simulink model "exo_df"  (R2018a)
settings: Solver=FixedStepDiscrete  StartTime=0.0  StopTime=inf  FixedStep=0.001  RelTol=1e-3  EnableMultiTasking=on
InitFcn:
  | init
values from neighbouring files (symbols this model uses):
  motor_saturation_torque = [10.0, 10.0]    [init.m]
  n = 2    [init.m]
  treadmillSpeed = 1.1    [init.m]
undefined symbols (not defined in the file or in its folder): DiscIntNeverNeededParam, Q8, USB
libraries: hdlsllib x50, quarc_library x16, dspsigops x2
(part 1 of 2)
settings Model: SimulationMode=external  ExtModeTrigDuration=2000000  Creator=mdmancho  LastModifiedBy=mdmancho
settings SolverCC: PositivePriorityOrder=on
settings RTWCC: SystemTargetFile=quarc_win64.tlc  TemplateMakefile=quarc_default_tmf  Description=QUARC Win64 Target
settings STFCustomTargetCC: TargetPreCompLibLocation=C:\PROGRA~3\QUARC\lib\2018a\win64\release  TargetLangStandard=C99 (ISO)  ConcurrentExecutionCompliant=on  SystemTargetFile=quarc_win64.tlc
settings GRTTargetCC: TargetPreCompLibLocation=C:\PROGRA~3\QUARC\lib\2018a\win64\release  ParMdlRefBuildCompliant=off  CompOptLevelCompliant=off  CombineOutputUpdateFcns=off  MatFileLogging=off  CPPClassGenCompliant=off  GRTInterface=on  UseToolchainInfoCompliant=off  ExtMode=on  ExtModeMexFile=quarc_comm

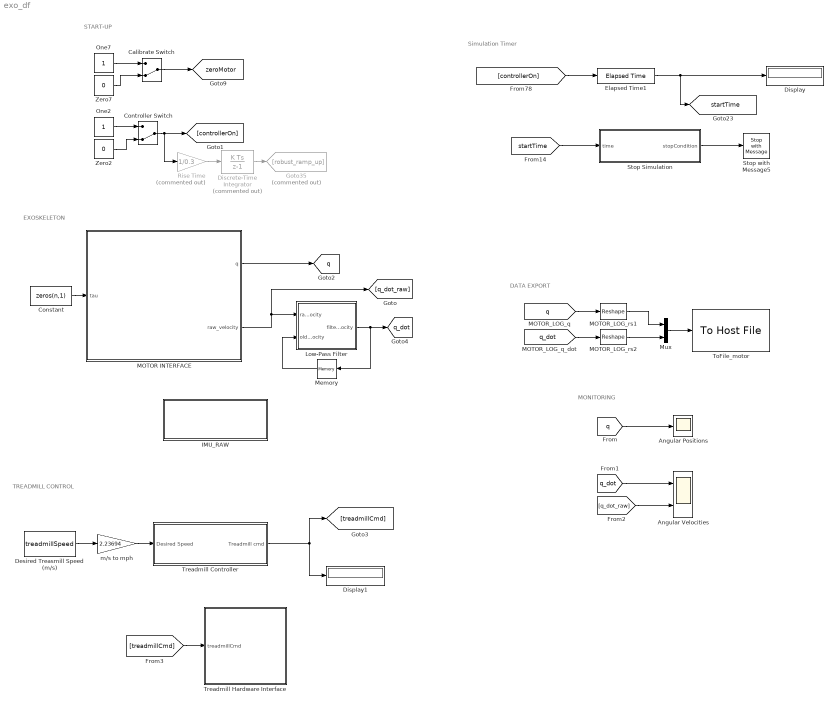
== system exo_df ==
  note: DATA EXPORT
  note: MONITORING
  note: START-UP
  note: EXOSKELETON
  note: Simulation Timer
  note: TREADMILL CONTROL
  Angular Positions : Scope
  Angular Velocities : Scope  NumInputPorts=2
  Calibrate Switch : ManualSwitch  CurrentSetting=0
  Constant : Constant  Value=zeros(n,1)
  Controller Switch : ManualSwitch  CurrentSetting=0
  Desired Treasmill Speed (m/s) : Constant  Value=treadmillSpeed
  Discrete-Time Integrator : DiscreteIntegrator  Commented=on  SampleTime=-1  LimitOutput=on  UpperSaturationLimit=1  LowerSaturationLimit=0  ICPrevOutput=DiscIntNeverNeededParam  ICPrevScaledInput=DiscIntNeverNeededParam
  Display : Display
  Display1 : Display
  Elapsed Time1 : quarc_library/Advanced/Timing/Elapsed Time  start_src=on
      settings: SourceProductName=QUARC Targets
  Goto35 : Goto  Commented=on  GotoTag=robust_ramp_up
  IMU_RAW : Subsystem  Description=Shoe VN-100 raw acquisition for OFFLINE validation only. No outports: nothing in the controller or the phase estimator may read it. See README.md.
  Low-Pass Filter : MATLAB Function  TreatAsAtomicUnit=on
  MOTOR INTERFACE : Subsystem
  MOTOR_LOG_rs1 : Reshape
  MOTOR_LOG_rs2 : Reshape
  Memory : quarc_library/Discrete/Memory  initial_condition=zeros(2,1)  sample_time=-1
      settings: SourceProductName=QUARC Targets
  Mux : Mux  Inputs=2
  One2 : Constant
  One7 : Constant
  Rise Time : Gain  Commented=on  Gain=1/0.3
  Stop Simulation : MATLAB Function  TreatAsAtomicUnit=on
  Stop with Message5 : quarc_library/Sinks/Error Handling/Stop with Message  message_type=Fixed error message  message_icon=Error  message=Simulation has ended
  ToFile_motor : quarc_library/Sinks/To Host/To Host File  file_name=C:\exo_logs\%{vn_log_run}_motor.mat  variable_name=motor  decimation=1  sample_time=-1  file_format=MAT-file v.5  options=No header or footer  append=off  final_file_name=C:\exo_logs\S02_T02_motor.mat  bitrate=2000000
  Treadmill Controller : Subsystem
  Treadmill Hardware Interface : Subsystem
  Zero2 : Constant  Value=0
  Zero7 : Constant  Value=0
  m/s to mph : Gain  Gain=2.23694
  tag scope: q=global, q_dot=global, startTime=global, zeroMotor=global
  wires:
  Memory/1 -> Low-Pass Filter/2(old_filtered_velocity)
  Low-Pass Filter/1(filtered_velocity) -> [q_dot], Memory/1
  MOTOR INTERFACE/2(raw_velocity) -> [q_dot_raw], Low-Pass Filter/1(raw_velocity)
  MOTOR INTERFACE/1(q) -> [q]
  [controllerOn] -> Elapsed Time1/1
  Elapsed Time1/1 -> Display/1, [startTime]
  Rise Time/1 -> Discrete-Time Integrator/1
  Discrete-Time Integrator/1 -> Goto35/1
  Calibrate Switch/1 -> [zeroMotor]
  Controller Switch/1 -> Rise Time/1, [controllerOn]
  One7/1 -> Calibrate Switch/1
  Zero2/1 -> Controller Switch/2
  Zero7/1 -> Calibrate Switch/2
  One2/1 -> Controller Switch/1
  Constant/1 -> MOTOR INTERFACE/1("tau ")
  [q] -> Angular Positions/1
  [q_dot] -> Angular Velocities/1
  [q_dot_raw] -> Angular Velocities/2
  [q] -> MOTOR_LOG_rs1/1
  [q_dot] -> MOTOR_LOG_rs2/1
  MOTOR_LOG_rs1/1 -> Mux/1
  MOTOR_LOG_rs2/1 -> Mux/2
  Mux/1 -> ToFile_motor/1
  [startTime] -> Stop Simulation/1(time)
  Stop Simulation/1(stopCondition) -> Stop with Message5/1
  [treadmillCmd] -> Treadmill Hardware Interface/1(treadmillCmd)
  Desired Treasmill Speed (m/s)/1 -> m/s to mph/1
  Treadmill Controller/1(Treadmill cmd) -> [treadmillCmd], Display1/1
  m/s to mph/1 -> Treadmill Controller/1(Desired Speed)

== system exo_df/IMU_RAW ==
  CLK : Subsystem
  RX : Subsystem

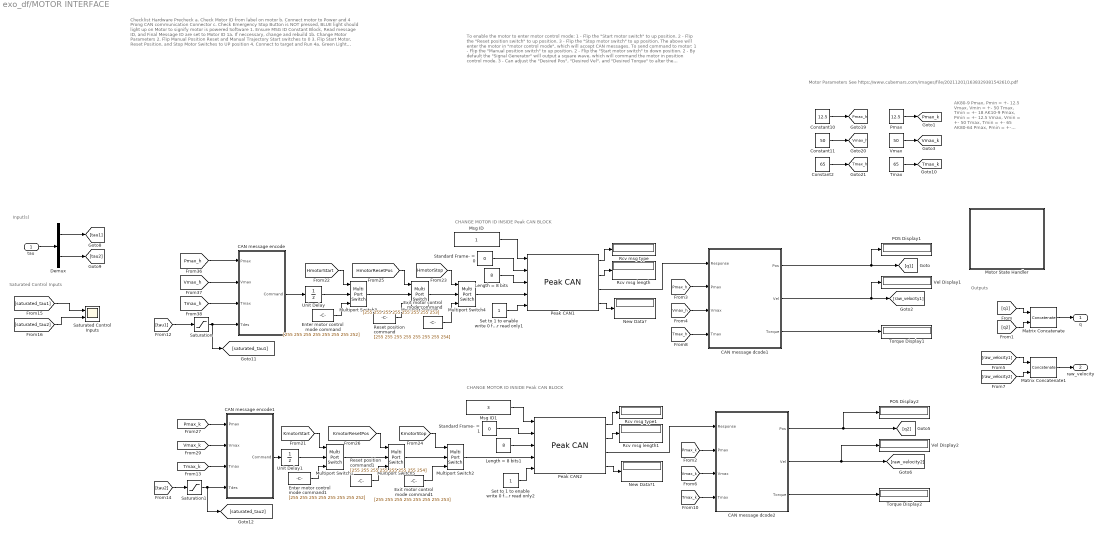
== system exo_df/MOTOR INTERFACE ==
  note: Saturated Control Inputs
  note: Input(s)
  note: Outputs
  note: CHANGE MOTOR ID INSIDE Peak CAN BLOCK
  note: Motor Parameters
      | See https://www.cubemars.com/images/file/20211201/1638329381542610.pdf
  note: To enable the motor to enter motor control mode:
      | 1 - Flip the "Start motor switch" to up position.
      | 2 - Flip the "Reset position switch" to up position.
      | 3 - Flip the "Stop motor switch" to up position.
      | The above will enter the motor in "motor control mode", which will accept CAN messages.
      |
      | To send command to motor:
      | 1 - Flip the "Manual position switch" to up position.
      | 2 - Flip the "Start motor switch" to down position.
      | 2 - By default the "Signal Generator" will output a square wave, which will command the motor in position control mode.
      | 3 - Can adjust the "Desired Pos", "Desired Vel", and "Desired Torque" to alter the command.
      | 4 - Can adjust the "Kp" and "Kd" to alter the P and D gain of the motor's internal controller.
      | 5 - If want to reset the motor position to 0, flip the "Reset position switch" to down position.
      |
      | To stop the motor and disable motor control mode:
      | 1 - Set the "Desired Pos", "Desired Vel", and "Desired Torque" to 0.
      | 2 - Flip the "Start motor switch" to up position.
      | 3 - Flip the "Stop motor switch" to down position.
  note: AK80-9
      | Pmax, Pmin = +- 12.5
      | Vmax, Vmin = +- 50
      | Tmax, Tmin = +- 18
      |
      | AK10-9
      | Pmax, Pmin = +- 12.5
      | Vmax, Vmin = +- 50
      | Tmax, Tmin = +- 65
      |
      | AK80-64
      | Pmax, Pmin = +- 12.5
      | Vmax, Vmin = +- 8
      | Tmax, Tmin = +- 144
  note: Checklist
      | Hardware Precheck
      | 	a. Check Motor ID from label on motor
      | 	b. Connect motor to Power and 4 Prong CAN communication Connector
      | 	c. Check Emergency Stop Button is NOT pressed, BLUE light should light up on Motor to 						signify motor is powered
      | Software
      | 1. Ensure MSG ID Constant Block, Read message ID, and Final Message ID are set to Motor ID
      | 	1a. If neccessary, change and rebuild
      | 	1b. Change Motor Parameters
      | 2. Flip Manual Position Reset and Manual Trajectory Start switches to 0
      | 3. Flip Start Motor, Reset Position, and Stop Motor Switches to UP position
      | 4. Connect to target and Run
      | 	4a. Green Light should light up on motor
      | 5. Flip Reset Position Switch to DOWN position, POS Display should now show a number (likely ~0 or ~-25)
      | 	5a. Flip Manual Position Offset switch, POS Display should now be 0
      | 	5b. Flip Reset Position Switch to UP position
      | 6. Flip Start Motor Switch to DOWN position
      | 7. Flip Manual Traj Start switch to 1
  note: CHANGE MOTOR ID INSIDE Peak CAN BLOCK
  "tau " : Inport
  CAN message dcode1 : Subsystem
  CAN message dcode2 : Subsystem
  CAN message encode : Subsystem
  CAN message encode1 : Subsystem
  Constant10 : Constant  Value=12.5
  Constant11 : Constant  Value=50
  Constant2 : Constant  Value=65
  Demux : Demux  Outputs=2
  Enter motor control mode command : Constant  Value=[255 255 255 255 255 255 255 252]  OutDataTypeStr=uint8
  Enter motor control mode command1 : Constant  Value=[255 255 255 255 255 255 255 252]  OutDataTypeStr=uint8
  Exit motor control mode command : Constant  Value=[255 255 255 255 255 255 255 253]  OutDataTypeStr=uint8
  Exit motor control mode command1 : Constant  Value=[255 255 255 255 255 255 255 253]  OutDataTypeStr=uint8
  Length = 8 bits : Constant  Value=8  OutDataTypeStr=uint8
  Length = 8 bits1 : Constant  Value=8  OutDataTypeStr=uint8
  Matrix Concatenate : Concatenate  Mode=Multidimensional array
  Matrix Concatenate1 : Concatenate  Mode=Multidimensional array
  Motor State Handler : Subsystem
  Msg ID : Constant  OutDataTypeStr=uint32
  Msg ID1 : Constant  Value=3  OutDataTypeStr=uint32
  Multiport Switch{1..6} (6 alike) : MultiPortSwitch  Inputs=2
  New Data? : Display
  New Data?1 : Display
  POS Display1 : Display
      settings: Format=decimal (Stored Integer)
  POS Display2 : Display
      settings: Format=decimal (Stored Integer)
  Peak CAN1 : quarc_library/Devices/Third-Party/Peak System/CAN Interfaces/Peak CAN  channel=2  device_type=PCAN-USB and PCAN-USB Pro  baud=1 Mbit/s  msg_ids=1  rcv_thread=off  thread_priority=0  send_final_message=on  final_id=1  final_type=0  final_data=[255 255 255 255 255 255 255 253]  sample_time=qc_get_step_size
      settings: SourceProductName=QUARC Targets
  Peak CAN2 : quarc_library/Devices/Third-Party/Peak System/CAN Interfaces/Peak CAN  channel=1  device_type=PCAN-USB and PCAN-USB Pro  baud=1 Mbit/s  msg_ids=3  rcv_thread=off  thread_priority=0  send_final_message=on  final_id=3  final_type=0  final_data=[255 255 255 255 255 255 255 253]  sample_time=qc_get_step_size
      settings: SourceProductName=QUARC Targets
  Pmax : Constant  Value=12.5
  Rcv msg length : Display
  Rcv msg length1 : Display
  Rcv msg type : Display
  Rcv msg type1 : Display
  Reset position command : Constant  Value=[255 255 255 255 255 255 255 254]  OutDataTypeStr=uint8
  Reset position command1 : Constant  Value=[255 255 255 255 255 255 255 254]  OutDataTypeStr=uint8
  Saturated Control Inputs : Scope  NumInputPorts=2
  Saturation : Saturate  UpperLimit=motor_saturation_torque(1)  LowerLimit=-motor_saturation_torque(1)
  Saturation1 : Saturate  UpperLimit=motor_saturation_torque(2)  LowerLimit=-motor_saturation_torque(2)
  Set to 1 to enable write 0 for read only1 : Constant  OutDataTypeStr=boolean
  Set to 1 to enable write 0 for read only2 : Constant  OutDataTypeStr=boolean
  Standard Frame- = 0 : Constant  Value=0  OutDataTypeStr=uint8
  Standard Frame- = 1 : Constant  Value=0  OutDataTypeStr=uint8
  Tmax : Constant  Value=65
  Torque Display1 : Display
      settings: Format=decimal (Stored Integer)
  Torque Display2 : Display
      settings: Format=decimal (Stored Integer)
  Unit Delay : UnitDelay  SampleTime=-1
  Unit Delay1 : UnitDelay  SampleTime=-1
  Vel Display1 : Display
      settings: Format=decimal (Stored Integer)
  Vel Display2 : Display
      settings: Format=decimal (Stored Integer)
  Vmax : Constant  Value=50
  q : Outport
  raw_velocity : Outport  Port=2
  tag scope: Pmax_h=global, Pmax_k=global, Tmax_h=global, Tmax_k=global, Vmax_h=global, Vmax_k=global
  wires:
  [Vmax_h] -> CAN message dcode1/3(Vmax)
  Saturation/1 -> [saturated_tau1], CAN message encode/4(Tdes)
  Length = 8 bits1/1 -> Peak CAN2/3
  Enter motor control mode command/1 -> Multiport Switch3/3
  [KmotorStart] -> Multiport Switch1/1
  [Pmax_h] -> CAN message encode/1(Pmax)
  Multiport Switch6/1 -> Multiport Switch4/2
  Msg ID1/1 -> Peak CAN2/1
  Peak CAN2/1 -> Rcv msg type1/1
  Multiport Switch2/1 -> Peak CAN2/4
  CAN message encode1/1(Command) -> Unit Delay1/1
  [HmotorStop] -> Multiport Switch4/1
  Unit Delay1/1 -> Multiport Switch1/2
  [Tmax_k] -> CAN message encode1/3(Tmax)
  Peak CAN2/4 -> New Data?1/1
  Multiport Switch4/1 -> Peak CAN1/4
  [Vmax_k] -> CAN message encode1/2(Vmax)
  [HmotorResetPos] -> Multiport Switch6/1
  Standard Frame- = 1/1 -> Peak CAN2/2
  Exit motor control mode command/1 -> Multiport Switch4/3
  Saturation1/1 -> [saturated_tau2], CAN message encode1/4(Tdes)
  [Tmax_h] -> CAN message dcode1/4(Tmax)
  Msg ID/1 -> Peak CAN1/1
  Peak CAN1/2 -> Rcv msg length/1
  Peak CAN1/1 -> Rcv msg type/1
  Multiport Switch3/1 -> Multiport Switch6/2
  [HmotorStart] -> Multiport Switch3/1
  [Tmax_h] -> CAN message encode/3(Tmax)
  Reset position command/1 -> Multiport Switch6/3
  Length = 8 bits/1 -> Peak CAN1/3
  Reset position command1/1 -> Multiport Switch5/3
  Unit Delay/1 -> Multiport Switch3/2
  Multiport Switch5/1 -> Multiport Switch2/2
  Standard Frame- = 0/1 -> Peak CAN1/2
  Peak CAN1/4 -> New Data?/1
  Peak CAN2/2 -> Rcv msg length1/1
  [Vmax_k] -> CAN message dcode2/3(Vmax)
  Multiport Switch1/1 -> Multiport Switch5/2
  Peak CAN1/3 -> CAN message dcode1/1(Response)
  CAN message encode/1(Command) -> Unit Delay/1
  Exit motor control mode command1/1 -> Multiport Switch2/3
  [Pmax_h] -> CAN message dcode1/2(Pmax)
  [KmotorResetPos] -> Multiport Switch5/1
  Enter motor control mode command1/1 -> Multiport Switch1/3
  [Vmax_h] -> CAN message encode/2(Vmax)
  [KmotorStop] -> Multiport Switch2/1
  [Pmax_k] -> CAN message dcode2/2(Pmax)
  Peak CAN2/3 -> CAN message dcode2/1(Response)
  [Tmax_k] -> CAN message dcode2/4(Tmax)
  [Pmax_k] -> CAN message encode1/1(Pmax)
  Set to 1 to enable write 0 for read only2/1 -> Peak CAN2/5
  Set to 1 to enable write 0 for read only1/1 -> Peak CAN1/5
  CAN message dcode1/1(Pos) -> [q1], POS Display1/1
  CAN message dcode1/2(Vel) -> [raw_velocity1], Vel Display1/1
  CAN message dcode2/1(Pos) -> [q2], POS Display2/1
  CAN message dcode2/2(Vel) -> [raw_velocity2], Vel Display2/1
  Constant10/1 -> [Pmax_h]
  Constant2/1 -> [Tmax_h]
  Vmax/1 -> [Vmax_k]
  Pmax/1 -> [Pmax_k]
  Constant11/1 -> [Vmax_h]
  Tmax/1 -> [Tmax_k]
  CAN message dcode2/3(Torque) -> Torque Display2/1
  CAN message dcode1/3(Torque) -> Torque Display1/1
  Matrix Concatenate/1 -> q/1
  [tau1] -> Saturation/1
  [tau2] -> Saturation1/1
  "tau "/1 -> Demux/1
  Demux/1 -> [tau1]
  Demux/2 -> [tau2]
  [q1] -> Matrix Concatenate/1
  [q2] -> Matrix Concatenate/2
  [raw_velocity1] -> Matrix Concatenate1/1
  [raw_velocity2] -> Matrix Concatenate1/2
  Matrix Concatenate1/1 -> raw_velocity/1
  [saturated_tau1] -> Saturated Control Inputs/1
  [saturated_tau2] -> Saturated Control Inputs/2

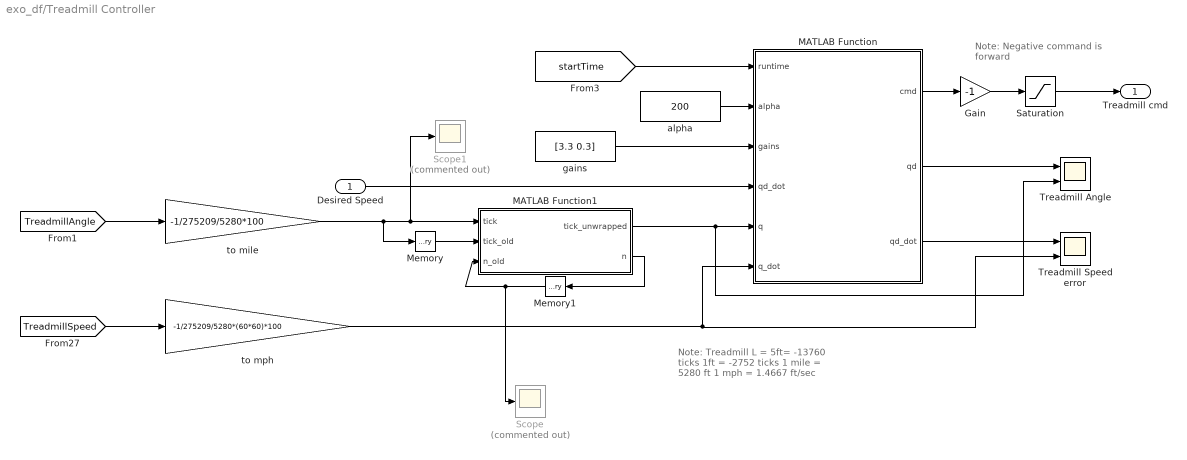
== system exo_df/Treadmill Controller ==
  note: Note:
      | Treadmill L = 5ft= -13760 ticks
      | 1ft = -2752 ticks
      | 1 mile = 5280 ft
      | 1 mph = 1.4667 ft/sec
  note: Note:
      | Negative command is forward
  Desired Speed : Inport
  Gain : Gain  Gain=-1
  MATLAB Function : MATLAB Function  TreatAsAtomicUnit=on
  MATLAB Function1 : MATLAB Function  TreatAsAtomicUnit=on
  Memory : Memory
  Memory1 : Memory
  Saturation : Saturate  UpperLimit=0  LowerLimit=-2
  Scope : Scope  Commented=on
  Scope1 : Scope  Commented=on
  Treadmill Angle : Scope  NumInputPorts=2
  Treadmill Speed error : Scope  NumInputPorts=2
  alpha : Constant  Value=200
  gains : Constant  Value=[3.3 0.3]
  to mile : Gain  Gain=-1/275209/5280*100
  to mph : Gain  Gain=-1/275209/5280*(60*60)*100
  Treadmill cmd : Outport
  wires:
  [TreadmillSpeed] -> to mph/1
  Saturation/1 -> Treadmill cmd/1
  to mph/1 -> Treadmill Speed error/2, MATLAB Function/6(q_dot)
  [startTime] -> MATLAB Function/1(runtime)
  gains/1 -> MATLAB Function/3(gains)
  MATLAB Function/1(cmd) -> Gain/1
  Desired Speed/1 -> MATLAB Function/4("qd_dot ")
  Gain/1 -> Saturation/1
  MATLAB Function/2(qd) -> Treadmill Angle/1
  MATLAB Function/3(qd_dot) -> Treadmill Speed error/1
  alpha/1 -> MATLAB Function/2(alpha)
  [TreadmillAngle] -> to mile/1
  Memory/1 -> MATLAB Function1/2(tick_old)
  MATLAB Function1/2(n) -> Memory1/1
  Memory1/1 -> Scope/1, MATLAB Function1/3(n_old)
  to mile/1 -> Memory/1, Scope1/1, MATLAB Function1/1(tick)
  MATLAB Function1/1(tick_unwrapped) -> Treadmill Angle/2, MATLAB Function/5(q)

== system exo_df/Treadmill Hardware Interface ==
  treadmillCmd : Inport
  Discrete Second-Order Low-Pass Filter2 : quarc_library/Discrete/Discrete Second-Order Low-Pass Filter  params_source=Internal (dialog parameters)  input_width=30  input_zeta=1  input_init=0  sample_time=sample_time
      settings: SourceProductName=QUARC Targets
  HIL Initialize : quarc_library/Data Acquisition/Generic/Configuration/HIL Initialize  Commented=on  object_name=QPID_e  board_type=qpid_e  board_number=0  board_options=enc0_dir=0;enc0_filter=1;enc0_a=1;enc0_b=1;enc0_z=0;enc0_reload=0;enc1_dir=0;enc1_filter=1;enc1_a=1;enc1_b=1;enc1_z=0;enc1_reload=0;enc2_dir=0;enc2_filter=1;enc2_a=1;enc2_b=1;enc2_z=0;enc2_reload=0;enc3_dir=0;enc3_filter=1;enc3_a=1;enc3_b=1;enc3_z=0;enc3_reload=0;enc4_dir=0;enc4_filter=1;enc4_a=1;enc4_b=1;enc4_z=0;enc4_reload=0;enc5_dir=0;enc5_filter=1;enc5_a=1;enc5_b=1;enc5_z=0;enc5_reload=0;enc6_dir=0;enc6_filter=1;enc6_a=1;enc6_b=1;enc6_z=0;enc6_reload=0;enc7_dir=0;enc7_filter=1;enc7_a=1;enc7_b=1;enc7_z=0;enc7_reload=0;ext_int_polarity=0;fuse_polarity=0;convert_polarity=0;watchdog_polarity=0;ext_int_watchdog=0;fuse_watchdog=0;trig1_watchdog=0;watchdog_to_trig1=0;watchdog_to_trig2=0;counter_to_trig0=0;trigger_adcs=0;latch_on_adc=0;pwm_immediate=0  exclusive=off  active=on  hardware_clocks=[0:16]  clock_modes=[]  initial_clock_frequencies=[]  set_clock_params_at_start=off  set_clock_params_at_switch_in=off  set_clock_frequencies_at_start=off  set_clock_frequencies_at_switch_in=off  analog_input_channels=[0:7]  analog_input_configurations=[]  analog_input_maximums=10  analog_input_minimums=-10  set_analog_input_params_at_start=off  set_analog_input_params_at_switch_in=off  analog_output_channels=[0:7]  analog_output_maximums=10  analog_output_minimums=-10  initial_analog_outputs=[0]  final_analog_outputs=[0]  watchdog_analog_outputs=0  set_analog_output_params_at_start=off  set_analog_output_params_at_switch_in=off  set_analog_outputs_at_start=on  set_analog_outputs_at_switch_in=off  set_analog_outputs_at_terminate=on  set_analog_outputs_at_switch_out=off  set_analog_outputs_on_watchdog=off  digital_input_channels=[]  digital_output_channels=[0:15]  digital_output_configuration=[]  initial_digital_outputs=[1]  final_digital_outputs=[1]  watchdog_digital_outputs=[2]  set_digital_output_params_at_start=off  set_digital_output_params_at_switch_in=off  set_digital_outputs_at_start=on  set_digital_outputs_at_switch_in=off  set_digital_outputs_at_terminate=on  set_digital_outputs_at_switch_out=off  set_digital_outputs_on_watchdog=off  encoder_channels=[0:7]  quadrature=[4]  encoder_filter_frequency=40e6/1  initial_encoder_counts=[0]  set_encoder_params_at_start=on  set_encoder_params_at_switch_in=off  set_encoder_counts_at_start=on  set_encoder_counts_at_switch_in=off  pwm_channels=[0:7]  pwm_modes=0  pwm_frequency=40e6/4096  pwm_configuration=[0]  pwm_alignment=[0]  pwm_polarity=[1]  pwm_leading_deadband=[0]  pwm_trailing_deadband=[0]  initial_pwm_outputs=[0]  final_pwm_outputs=[0]  watchdog_pwm_outputs=[0]  set_pwm_params_at_start=on  set_pwm_params_at_switch_in=off  set_pwm_outputs_at_start=on  set_pwm_outputs_at_switch_in=off  set_pwm_outputs_at_terminate=on  set_pwm_outputs_at_switch_out=off  set_pwm_outputs_on_watchdog=off  other_output_channels=[]  initial_other_outputs=[]  final_other_outputs=[]  watchdog_other_outputs=[]  set_other_outputs_at_start=off  set_other_outputs_at_switch_in=off  set_other_outputs_at_terminate=off  set_other_outputs_at_switch_out=off  set_other_outputs_on_watchdog=off
  HIL Initialize1 : quarc_library/Data Acquisition/Generic/Configuration/HIL Initialize  object_name=Q8-USB  board_type=q8_usb  board_number=0  board_options=update_rate=normal;decimation=1  exclusive=off  active=on  hardware_clocks=[0:2]  clock_modes=[]  initial_clock_frequencies=[]  set_clock_params_at_start=off  set_clock_params_at_switch_in=off  set_clock_frequencies_at_start=off  set_clock_frequencies_at_switch_in=off  analog_input_channels=[0:7]  analog_input_configurations=[]  analog_input_maximums=10  analog_input_minimums=-10  set_analog_input_params_at_start=on  set_analog_input_params_at_switch_in=off  analog_output_channels=[0:7]  analog_output_maximums=10  analog_output_minimums=-10  initial_analog_outputs=[0]  final_analog_outputs=[0]  watchdog_analog_outputs=0  set_analog_output_params_at_start=on  set_analog_output_params_at_switch_in=off  set_analog_outputs_at_start=on  set_analog_outputs_at_switch_in=off  set_analog_outputs_at_terminate=on  set_analog_outputs_at_switch_out=off  set_analog_outputs_on_watchdog=off  digital_input_channels=[]  digital_output_channels=[0]  digital_output_configuration=[]  initial_digital_outputs=[1]  final_digital_outputs=[1]  watchdog_digital_outputs=[0]  set_digital_output_params_at_start=off  set_digital_output_params_at_switch_in=off  set_digital_outputs_at_start=on  set_digital_outputs_at_switch_in=off  set_digital_outputs_at_terminate=on  set_digital_outputs_at_switch_out=off  set_digital_outputs_on_watchdog=off  encoder_channels=[0:7]  quadrature=[4]  encoder_filter_frequency=[]  initial_encoder_counts=[0]  set_encoder_params_at_start=on  set_encoder_params_at_switch_in=off  set_encoder_counts_at_start=on  set_encoder_counts_at_switch_in=off  pwm_channels=[0:7]  pwm_modes=0  pwm_frequency=99.532799999999995e6/4095  pwm_configuration=[0]  pwm_alignment=[0]  pwm_polarity=[1]  pwm_leading_deadband=[0]  pwm_trailing_deadband=[0]  initial_pwm_outputs=[0]  final_pwm_outputs=[0]  watchdog_pwm_outputs=[0]  set_pwm_params_at_start=on  set_pwm_params_at_switch_in=off  set_pwm_outputs_at_start=on  set_pwm_outputs_at_switch_in=off  set_pwm_outputs_at_terminate=on  set_pwm_outputs_at_switch_out=off  set_pwm_outputs_on_watchdog=off  other_output_channels=[]  initial_other_outputs=[]  final_other_outputs=[]  watchdog_other_outputs=[]  set_other_outputs_at_start=off  set_other_outputs_at_switch_in=off  set_other_outputs_at_terminate=off  set_other_outputs_at_switch_out=off  set_other_outputs_on_watchdog=off
  HIL Read2 : quarc_library/Data Acquisition/Generic/Immediate I//O/HIL Read  object_name=Q8-USB  analog_channels=[]  encoder_channels=[0]  digital_channels=[]  other_channels=[14000]  sample_time=sample_time  active=on  vector_output=off  data_type_mode=Inherit via back propagation  encoder_data_type=double  digital_data_type=boolean
  HIL Write : quarc_library/Data Acquisition/Generic/Immediate I//O/HIL Write  object_name=Q8-USB  analog_channels=0  pwm_channels=[]  digital_channels=[]  other_channels=[]  sample_time=sample_time  active=off  vector_input=off
  Motor Cmd to Quanser : Scope  NumInputPorts=2
  Scope : Scope
  tag scope: TreadmillAngle=global, TreadmillSpeed=global
  wires:
  Discrete Second-Order Low-Pass Filter2/1 -> [TreadmillSpeed]
  HIL Read2/2 -> Discrete Second-Order Low-Pass Filter2/1
  HIL Read2/1 -> [TreadmillAngle]
  [TreadmillAngle] -> Motor Cmd to Quanser/1
  [TreadmillSpeed] -> Motor Cmd to Quanser/2
  treadmillCmd/1 -> Scope/1, HIL Write/1

== system exo_df/IMU_RAW/CLK ==
  ToFile_clk : quarc_library/Sinks/To Host/To Host File  file_name=C:\exo_logs\%{vn_log_run}_clk.mat  variable_name=clk  decimation=1  sample_time=-1  file_format=MAT-file v.5  options=No header or footer  append=off  final_file_name=C:\exo_logs\S02_T02_clk.mat  bitrate=2000000
  qpc_clock : S-Function  FunctionName=qpc_clock  Parameters=0.001  SFunctionDeploymentMode=off  EnableBusSupport=off
  wires:
  qpc_clock/1 -> ToFile_clk/1  "qpc_s"

== system exo_df/IMU_RAW/RX ==
  DTC{2..8} (7 alike) : DataTypeConversion  OutDataTypeStr=double
  Mux : Mux  Inputs=7
  Term_bytes : Terminator
  ToFile_bytes : quarc_library/Sinks/To Host/To Host File  file_name=C:\exo_logs\%{vn_log_run}_imu_bytes.mat  variable_name=imu_bytes_p4  decimation=1  sample_time=-1  file_format=MAT-file v.5  options=No header or footer  append=off  final_file_name=C:\exo_logs\S02_T02_imu_bytes.mat  bitrate=2000000
  ToFile_diag : quarc_library/Sinks/To Host/To Host File  file_name=C:\exo_logs\%{vn_log_run}_imu_diag.mat  variable_name=imu_diag  decimation=1  sample_time=-1  file_format=MAT-file v.5  options=No header or footer  append=off  final_file_name=C:\exo_logs\S02_T02_imu_diag.mat  bitrate=2000000
  vn_raw_rx : S-Function  FunctionName=vn_raw_rx  Parameters=9, 921600, 0.002, 128  SFunctionDeploymentMode=off  EnableBusSupport=off
  wires:
  vn_raw_rx/1 -> Term_bytes/1  "imu_bytes"
  vn_raw_rx/9 -> ToFile_bytes/1  "imu_bytes_p4"
  vn_raw_rx/2 -> DTC2/1  "n_read"
  DTC2/1 -> Mux/1
  vn_raw_rx/3 -> DTC3/1  "t_rx_qpc"
  DTC3/1 -> Mux/2
  vn_raw_rx/4 -> DTC4/1  "queued"
  DTC4/1 -> Mux/3
  vn_raw_rx/5 -> DTC5/1  "cum_bytes"
  DTC5/1 -> Mux/4
  vn_raw_rx/6 -> DTC6/1  "err_calls"
  DTC6/1 -> Mux/5
  vn_raw_rx/7 -> DTC7/1  "err_mask"
  DTC7/1 -> Mux/6
  vn_raw_rx/8 -> DTC8/1  "dur_us"
  DTC8/1 -> Mux/7
  Mux/1 -> ToFile_diag/1

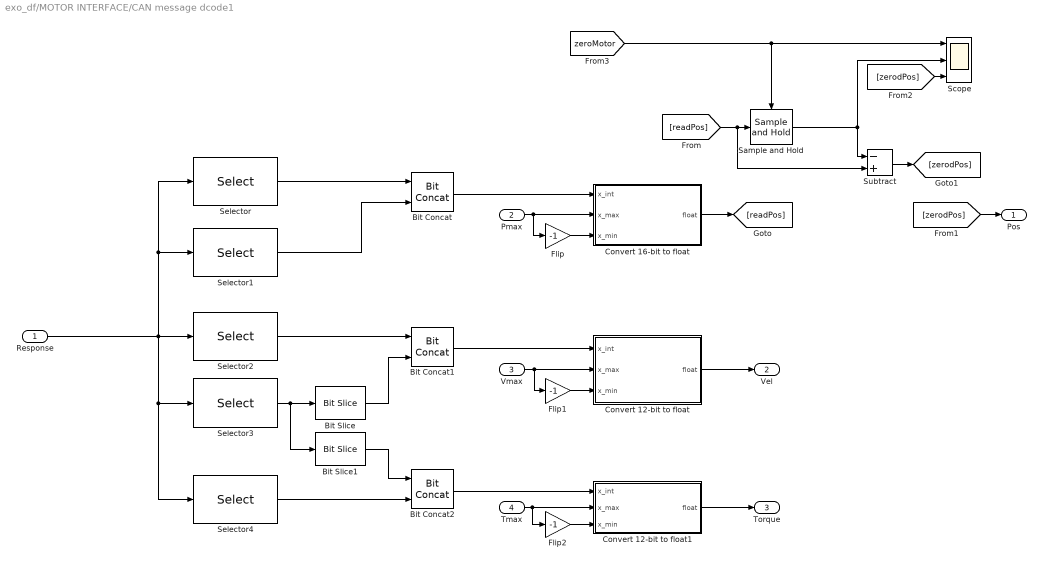
== system exo_df/MOTOR INTERFACE/CAN message dcode1 ==
  Response : Inport
  Pmax : Inport  Port=2
  Vmax : Inport  Port=3
  Tmax : Inport  Port=4
  Bit Concat : hdlsllib/Logic and Bit Operations/Bit Concat  numInputs=2
      settings: SourceProductName=HDL Coder  SourceProductBaseCode=HD
  Bit Concat1 : hdlsllib/Logic and Bit Operations/Bit Concat  numInputs=2
      settings: SourceProductName=HDL Coder  SourceProductBaseCode=HD
  Bit Concat2 : hdlsllib/Logic and Bit Operations/Bit Concat  numInputs=2
      settings: SourceProductName=HDL Coder  SourceProductBaseCode=HD
  Bit Slice : hdlsllib/Logic and Bit Operations/Bit Slice  lidx=7  ridx=4
  Bit Slice1 : hdlsllib/Logic and Bit Operations/Bit Slice  lidx=3  ridx=0
  Convert 12-bit to float : Subsystem
  Convert 12-bit to float1 : Subsystem
  Convert 16-bit to float : Subsystem
  Flip : Gain  Gain=-1
  Flip1 : Gain  Gain=-1
  Flip2 : Gain  Gain=-1
  Sample and Hold : dspsigops/Sample and Hold  trig=Rising edge  initCond=0  latchinput=off
  Scope : Scope  NumInputPorts=3
  Selector : Selector  IndexMode=Zero-based  InputPortWidth=8  IndexOptions=Index vector (dialog)  Indices=[1]  OutputSizes=1
  Selector1 : Selector  IndexMode=Zero-based  InputPortWidth=8  IndexOptions=Index vector (dialog)  Indices=[2]  OutputSizes=1
  Selector2 : Selector  IndexMode=Zero-based  InputPortWidth=8  IndexOptions=Index vector (dialog)  Indices=[3]  OutputSizes=1
  Selector3 : Selector  IndexMode=Zero-based  InputPortWidth=8  IndexOptions=Index vector (dialog)  Indices=[4]  OutputSizes=1
  Selector4 : Selector  IndexMode=Zero-based  InputPortWidth=8  IndexOptions=Index vector (dialog)  Indices=[5]  OutputSizes=1
  Subtract : Sum  Inputs=-+
  Pos : Outport  VectorParamsAs1DForOutWhenUnconnected=on
  Vel : Outport  Port=2  VectorParamsAs1DForOutWhenUnconnected=on
  Torque : Outport  Port=3  VectorParamsAs1DForOutWhenUnconnected=on
  wires:
  Vmax/1 -> Flip1/1, Convert 12-bit to float/2(x_max)
  Selector3/1 -> Bit Slice1/1, Bit Slice/1
  Bit Slice1/1 -> Bit Concat2/1
  Response/1 -> Selector4/1, Selector3/1, Selector/1, Selector1/1, Selector2/1
  Selector/1 -> Bit Concat/1
  Bit Concat2/1 -> Convert 12-bit to float1/1(x_int)
  Selector1/1 -> Bit Concat/2
  Pmax/1 -> Flip/1, Convert 16-bit to float/2(x_max)
  Bit Concat/1 -> Convert 16-bit to float/1(x_int)
  Selector2/1 -> Bit Concat1/1
  Selector4/1 -> Bit Concat2/2
  Flip1/1 -> Convert 12-bit to float/3(x_min)
  Tmax/1 -> Flip2/1, Convert 12-bit to float1/2(x_max)
  Bit Concat1/1 -> Convert 12-bit to float/1(x_int)
  Flip/1 -> Convert 16-bit to float/3(x_min)
  Bit Slice/1 -> Bit Concat1/2
  Convert 12-bit to float1/1(float) -> Torque/1
  Flip2/1 -> Convert 12-bit to float1/3(x_min)
  Convert 16-bit to float/1(float) -> [readPos]
  [readPos] -> Subtract/2, Sample and Hold/1
  Sample and Hold/1 -> Subtract/1, Scope/2
  Subtract/1 -> [zerodPos]
  [zerodPos] -> Pos/1
  [zerodPos] -> Scope/3
  [zeroMotor] -> Sample and Hold/Trigger, Scope/1
  Convert 12-bit to float/1(float) -> Vel/1

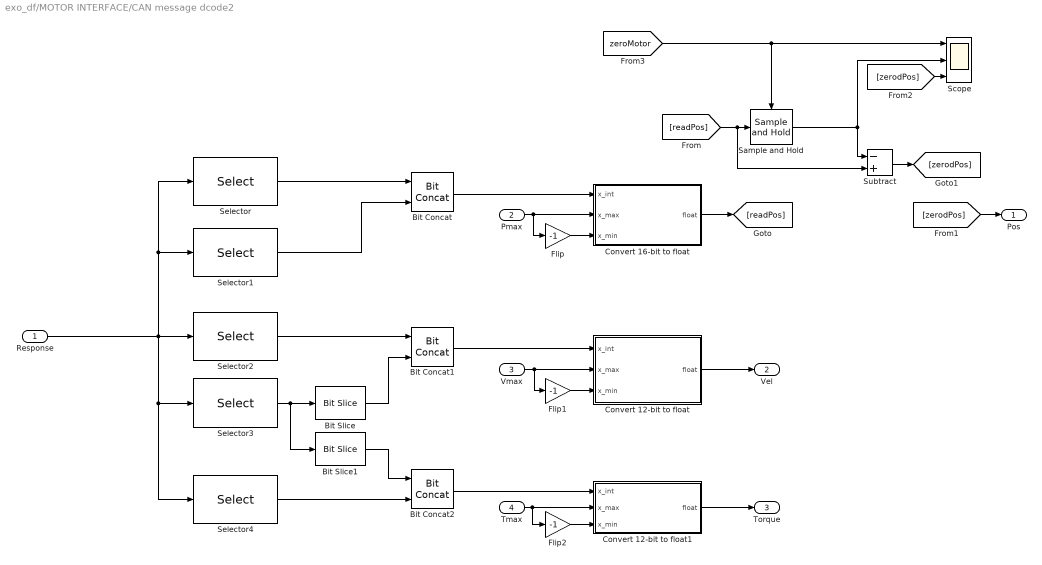
== system exo_df/MOTOR INTERFACE/CAN message dcode2 ==
  Response : Inport
  Pmax : Inport  Port=2
  Vmax : Inport  Port=3
  Tmax : Inport  Port=4
  Bit Concat : hdlsllib/Logic and Bit Operations/Bit Concat  numInputs=2
      settings: SourceProductName=HDL Coder  SourceProductBaseCode=HD
  Bit Concat1 : hdlsllib/Logic and Bit Operations/Bit Concat  numInputs=2
      settings: SourceProductName=HDL Coder  SourceProductBaseCode=HD
  Bit Concat2 : hdlsllib/Logic and Bit Operations/Bit Concat  numInputs=2
      settings: SourceProductName=HDL Coder  SourceProductBaseCode=HD
  Bit Slice : hdlsllib/Logic and Bit Operations/Bit Slice  lidx=7  ridx=4
  Bit Slice1 : hdlsllib/Logic and Bit Operations/Bit Slice  lidx=3  ridx=0
  Convert 12-bit to float : Subsystem
  Convert 12-bit to float1 : Subsystem
  Convert 16-bit to float : Subsystem
  Flip : Gain  Gain=-1
  Flip1 : Gain  Gain=-1
  Flip2 : Gain  Gain=-1
  Sample and Hold : dspsigops/Sample and Hold  trig=Rising edge  initCond=0  latchinput=off
  Scope : Scope  NumInputPorts=3
  Selector : Selector  IndexMode=Zero-based  InputPortWidth=8  IndexOptions=Index vector (dialog)  Indices=[1]  OutputSizes=1
  Selector1 : Selector  IndexMode=Zero-based  InputPortWidth=8  IndexOptions=Index vector (dialog)  Indices=[2]  OutputSizes=1
  Selector2 : Selector  IndexMode=Zero-based  InputPortWidth=8  IndexOptions=Index vector (dialog)  Indices=[3]  OutputSizes=1
  Selector3 : Selector  IndexMode=Zero-based  InputPortWidth=8  IndexOptions=Index vector (dialog)  Indices=[4]  OutputSizes=1
  Selector4 : Selector  IndexMode=Zero-based  InputPortWidth=8  IndexOptions=Index vector (dialog)  Indices=[5]  OutputSizes=1
  Subtract : Sum  Inputs=-+
  Pos : Outport  VectorParamsAs1DForOutWhenUnconnected=on
  Vel : Outport  Port=2  VectorParamsAs1DForOutWhenUnconnected=on
  Torque : Outport  Port=3  VectorParamsAs1DForOutWhenUnconnected=on
  wires:
  [zerodPos] -> Scope/3
  [zerodPos] -> Pos/1
  Subtract/1 -> [zerodPos]
  Sample and Hold/1 -> Scope/2, Subtract/1
  [readPos] -> Sample and Hold/1, Subtract/2
  Convert 16-bit to float/1(float) -> [readPos]
  Flip2/1 -> Convert 12-bit to float1/3(x_min)
  Convert 12-bit to float1/1(float) -> Torque/1
  Bit Slice/1 -> Bit Concat1/2
  Flip/1 -> Convert 16-bit to float/3(x_min)
  Bit Concat1/1 -> Convert 12-bit to float/1(x_int)
  Tmax/1 -> Convert 12-bit to float1/2(x_max), Flip2/1
  Flip1/1 -> Convert 12-bit to float/3(x_min)
  Selector4/1 -> Bit Concat2/2
  Selector2/1 -> Bit Concat1/1
  Bit Concat/1 -> Convert 16-bit to float/1(x_int)
  Pmax/1 -> Convert 16-bit to float/2(x_max), Flip/1
  Selector1/1 -> Bit Concat/2
  Bit Concat2/1 -> Convert 12-bit to float1/1(x_int)
  Selector/1 -> Bit Concat/1
  Response/1 -> Selector2/1, Selector1/1, Selector/1, Selector3/1, Selector4/1
  Bit Slice1/1 -> Bit Concat2/1
  Selector3/1 -> Bit Slice/1, Bit Slice1/1
  Vmax/1 -> Convert 12-bit to float/2(x_max), Flip1/1
  [zeroMotor] -> Sample and Hold/Trigger, Scope/1
  Convert 12-bit to float/1(float) -> Vel/1

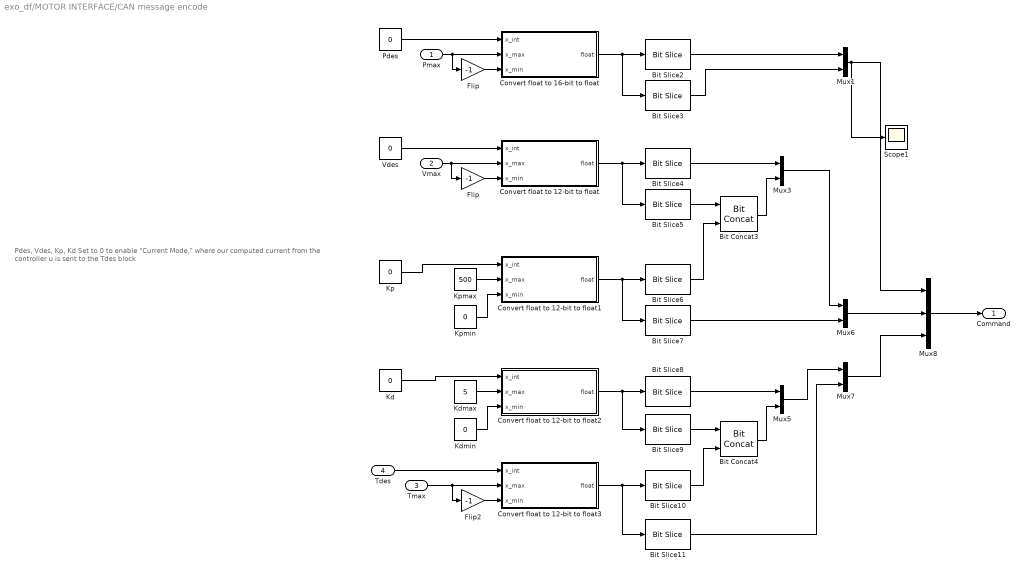
== system exo_df/MOTOR INTERFACE/CAN message encode ==
  note: Pdes, Vdes, Kp, Kd Set to 0 to enable "Current Mode," where our computed current from the controller u is sent to the Tdes block
  Pmax : Inport
  Vmax : Inport  Port=2
  Tmax : Inport  Port=3
  Tdes : Inport  Port=4
  Bit Concat3 : hdlsllib/Logic and Bit Operations/Bit Concat  numInputs=2
      settings: SourceProductName=HDL Coder  SourceProductBaseCode=HD
  Bit Concat4 : hdlsllib/Logic and Bit Operations/Bit Concat  numInputs=2
      settings: SourceProductName=HDL Coder  SourceProductBaseCode=HD
  Bit Slice10 : hdlsllib/Logic and Bit Operations/Bit Slice  lidx=11  ridx=8
  Bit Slice11 : hdlsllib/Logic and Bit Operations/Bit Slice  lidx=7  ridx=0
  Bit Slice2 : hdlsllib/Logic and Bit Operations/Bit Slice  lidx=15  ridx=8
  Bit Slice3 : hdlsllib/Logic and Bit Operations/Bit Slice  lidx=7  ridx=0
  Bit Slice4 : hdlsllib/Logic and Bit Operations/Bit Slice  lidx=11  ridx=4
  Bit Slice5 : hdlsllib/Logic and Bit Operations/Bit Slice  lidx=3  ridx=0
  Bit Slice6 : hdlsllib/Logic and Bit Operations/Bit Slice  lidx=11  ridx=8
  Bit Slice7 : hdlsllib/Logic and Bit Operations/Bit Slice  lidx=7  ridx=0
  Bit Slice8 : hdlsllib/Logic and Bit Operations/Bit Slice  lidx=11  ridx=4
  Bit Slice9 : hdlsllib/Logic and Bit Operations/Bit Slice  lidx=3  ridx=0
  Convert float to 12-bit to float : Subsystem
  Convert float to 12-bit to float1 : Subsystem
  Convert float to 12-bit to float2 : Subsystem
  Convert float to 12-bit to float3 : Subsystem
  Convert float to 16-bit to float : Subsystem
  Flip : Gain  Gain=-1
  "Flip " : Gain  Gain=-1
  Flip2 : Gain  Gain=-1
  Kd : Constant  Value=0
  Kdmax : Constant  Value=5
  Kdmin : Constant  Value=0
  Kp : Constant  Value=0
  Kpmax : Constant  Value=500
  Kpmin : Constant  Value=0
  Mux{1,3,5..7} (5 alike) : Mux  Inputs=2
  Mux8 : Mux  Inputs=3
  Pdes : Constant  Value=0
  Scope1 : Scope
  Vdes : Constant  Value=0
  Command : Outport  VectorParamsAs1DForOutWhenUnconnected=on
  wires:
  Bit Slice5/1 -> Bit Concat3/1
  "Flip "/1 -> Convert float to 16-bit to float/3(x_min)
  Bit Slice10/1 -> Bit Concat4/2
  Bit Slice9/1 -> Bit Concat4/1
  Flip/1 -> Convert float to 12-bit to float/3(x_min)
  Convert float to 12-bit to float3/1(float) -> Bit Slice11/1, Bit Slice10/1
  Vmax/1 -> Flip/1, Convert float to 12-bit to float/2(x_max)
  Mux7/1 -> Mux8/3
  Convert float to 12-bit to float/1(float) -> Bit Slice4/1, Bit Slice5/1
  Bit Slice7/1 -> Mux6/2
  Convert float to 12-bit to float2/1(float) -> Bit Slice9/1, Bit Slice8/1
  Bit Slice6/1 -> Bit Concat3/2
  Mux5/1 -> Mux7/1
  Mux8/1 -> Command/1
  Bit Slice4/1 -> Mux3/1
  Bit Concat4/1 -> Mux5/2
  Convert float to 16-bit to float/1(float) -> Bit Slice3/1, Bit Slice2/1
  Bit Slice2/1 -> Mux1/1
  Kdmax/1 -> Convert float to 12-bit to float2/2(x_max)
  Bit Slice8/1 -> Mux5/1
  Kdmin/1 -> Convert float to 12-bit to float2/3(x_min)
  Kpmax/1 -> Convert float to 12-bit to float1/2(x_max)
  Convert float to 12-bit to float1/1(float) -> Bit Slice7/1, Bit Slice6/1
  Mux1/1 -> Scope1/1, Mux8/1
  Bit Slice11/1 -> Mux7/2
  Bit Slice3/1 -> Mux1/2
  Pmax/1 -> "Flip "/1, Convert float to 16-bit to float/2(x_max)
  Mux6/1 -> Mux8/2
  Bit Concat3/1 -> Mux3/2
  Tmax/1 -> Flip2/1, Convert float to 12-bit to float3/2(x_max)
  Kpmin/1 -> Convert float to 12-bit to float1/3(x_min)
  Mux3/1 -> Mux6/1
  Flip2/1 -> Convert float to 12-bit to float3/3(x_min)
  Vdes/1 -> Convert float to 12-bit to float/1(x_int)
  Kd/1 -> Convert float to 12-bit to float2/1(x_int)
  Kp/1 -> Convert float to 12-bit to float1/1(x_int)
  Pdes/1 -> Convert float to 16-bit to float/1(x_int)
  Tdes/1 -> Convert float to 12-bit to float3/1(x_int)

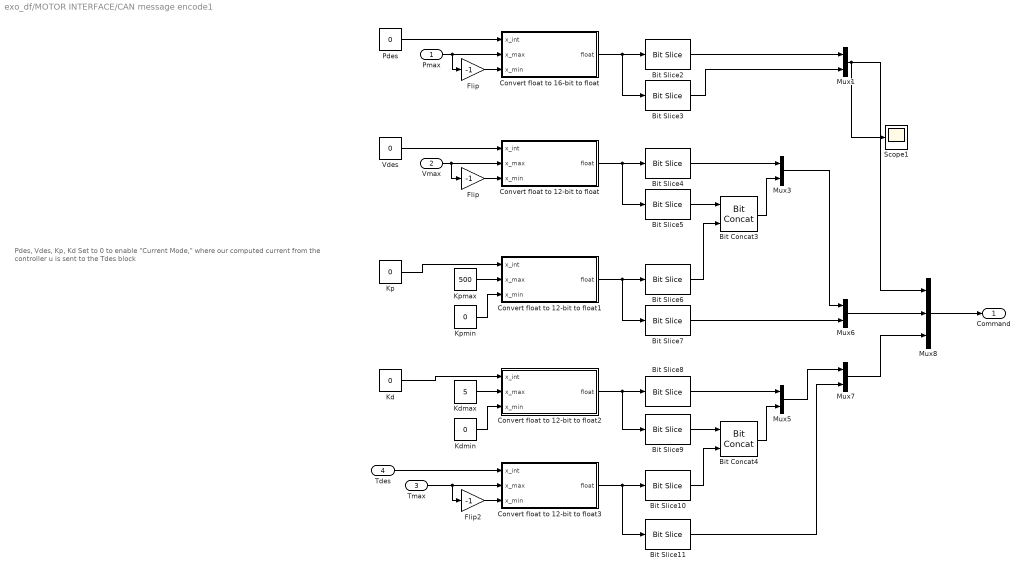
== system exo_df/MOTOR INTERFACE/CAN message encode1 ==
  note: Pdes, Vdes, Kp, Kd Set to 0 to enable "Current Mode," where our computed current from the controller u is sent to the Tdes block
  Pmax : Inport
  Vmax : Inport  Port=2
  Tmax : Inport  Port=3
  Tdes : Inport  Port=4
  Bit Concat3 : hdlsllib/Logic and Bit Operations/Bit Concat  numInputs=2
      settings: SourceProductName=HDL Coder  SourceProductBaseCode=HD
  Bit Concat4 : hdlsllib/Logic and Bit Operations/Bit Concat  numInputs=2
      settings: SourceProductName=HDL Coder  SourceProductBaseCode=HD
  Bit Slice10 : hdlsllib/Logic and Bit Operations/Bit Slice  lidx=11  ridx=8
  Bit Slice11 : hdlsllib/Logic and Bit Operations/Bit Slice  lidx=7  ridx=0
  Bit Slice2 : hdlsllib/Logic and Bit Operations/Bit Slice  lidx=15  ridx=8
  Bit Slice3 : hdlsllib/Logic and Bit Operations/Bit Slice  lidx=7  ridx=0
  Bit Slice4 : hdlsllib/Logic and Bit Operations/Bit Slice  lidx=11  ridx=4
  Bit Slice5 : hdlsllib/Logic and Bit Operations/Bit Slice  lidx=3  ridx=0
  Bit Slice6 : hdlsllib/Logic and Bit Operations/Bit Slice  lidx=11  ridx=8
  Bit Slice7 : hdlsllib/Logic and Bit Operations/Bit Slice  lidx=7  ridx=0
  Bit Slice8 : hdlsllib/Logic and Bit Operations/Bit Slice  lidx=11  ridx=4
  Bit Slice9 : hdlsllib/Logic and Bit Operations/Bit Slice  lidx=3  ridx=0
  Convert float to 12-bit to float : Subsystem
  Convert float to 12-bit to float1 : Subsystem
  Convert float to 12-bit to float2 : Subsystem
  Convert float to 12-bit to float3 : Subsystem
  Convert float to 16-bit to float : Subsystem
  Flip : Gain  Gain=-1
  "Flip " : Gain  Gain=-1
  Flip2 : Gain  Gain=-1
  Kd : Constant  Value=0
  Kdmax : Constant  Value=5
  Kdmin : Constant  Value=0
  Kp : Constant  Value=0
  Kpmax : Constant  Value=500
  Kpmin : Constant  Value=0
  Mux{1,3,5..7} (5 alike) : Mux  Inputs=2
  Mux8 : Mux  Inputs=3
  Pdes : Constant  Value=0
  Scope1 : Scope
  Vdes : Constant  Value=0
  Command : Outport  VectorParamsAs1DForOutWhenUnconnected=on
  wires:
  Tdes/1 -> Convert float to 12-bit to float3/1(x_int)
  Pdes/1 -> Convert float to 16-bit to float/1(x_int)
  Kp/1 -> Convert float to 12-bit to float1/1(x_int)
  Kd/1 -> Convert float to 12-bit to float2/1(x_int)
  Vdes/1 -> Convert float to 12-bit to float/1(x_int)
  Flip2/1 -> Convert float to 12-bit to float3/3(x_min)
  Mux3/1 -> Mux6/1
  Kpmin/1 -> Convert float to 12-bit to float1/3(x_min)
  Tmax/1 -> Convert float to 12-bit to float3/2(x_max), Flip2/1
  Bit Concat3/1 -> Mux3/2
  Mux6/1 -> Mux8/2
  Pmax/1 -> Convert float to 16-bit to float/2(x_max), "Flip "/1
  Bit Slice3/1 -> Mux1/2
  Bit Slice11/1 -> Mux7/2
  Mux1/1 -> Mux8/1, Scope1/1
  Convert float to 12-bit to float1/1(float) -> Bit Slice6/1, Bit Slice7/1
  Kpmax/1 -> Convert float to 12-bit to float1/2(x_max)
  Kdmin/1 -> Convert float to 12-bit to float2/3(x_min)
  Bit Slice8/1 -> Mux5/1
  Kdmax/1 -> Convert float to 12-bit to float2/2(x_max)
  Bit Slice2/1 -> Mux1/1
  Convert float to 16-bit to float/1(float) -> Bit Slice2/1, Bit Slice3/1
  Bit Concat4/1 -> Mux5/2
  Bit Slice4/1 -> Mux3/1
  Mux8/1 -> Command/1
  Mux5/1 -> Mux7/1
  Bit Slice6/1 -> Bit Concat3/2
  Convert float to 12-bit to float2/1(float) -> Bit Slice8/1, Bit Slice9/1
  Bit Slice7/1 -> Mux6/2
  Convert float to 12-bit to float/1(float) -> Bit Slice5/1, Bit Slice4/1
  Mux7/1 -> Mux8/3
  Vmax/1 -> Convert float to 12-bit to float/2(x_max), Flip/1
  Convert float to 12-bit to float3/1(float) -> Bit Slice10/1, Bit Slice11/1
  Flip/1 -> Convert float to 12-bit to float/3(x_min)
  Bit Slice9/1 -> Bit Concat4/1
  Bit Slice10/1 -> Bit Concat4/2
  "Flip "/1 -> Convert float to 16-bit to float/3(x_min)
  Bit Slice5/1 -> Bit Concat3/1

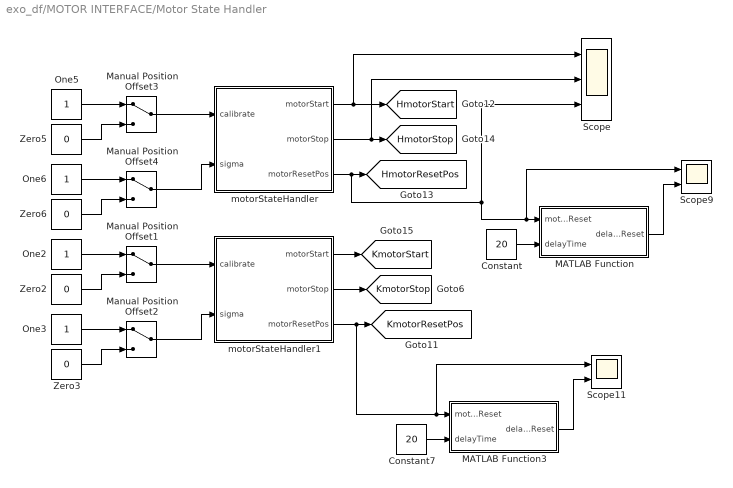
== system exo_df/MOTOR INTERFACE/Motor State Handler ==
  Constant : Constant  Value=20
  Constant7 : Constant  Value=20
  MATLAB Function : MATLAB Function  TreatAsAtomicUnit=on
  MATLAB Function3 : MATLAB Function  TreatAsAtomicUnit=on
  Manual Position Offset{1..4} (4 alike) : ManualSwitch
  One{2..3,5..6} (4 alike) : Constant
  Scope : Scope  NumInputPorts=3
  Scope11 : Scope  NumInputPorts=2
  Scope9 : Scope  NumInputPorts=2
  Zero{2..3,5..6} (4 alike) : Constant  Value=0
  motorStateHandler : MATLAB Function  TreatAsAtomicUnit=on
  motorStateHandler1 : MATLAB Function  TreatAsAtomicUnit=on
  tag scope: HmotorResetPos=global, HmotorStart=global, HmotorStop=global, KmotorResetPos=global, KmotorStart=global, KmotorStop=global
  wires:
  motorStateHandler1/2(motorStop) -> [KmotorStop]
  Zero3/1 -> Manual Position Offset2/2
  Manual Position Offset2/1 -> motorStateHandler1/2(sigma)
  motorStateHandler/3(motorResetPos) -> Scope9/1, MATLAB Function/1(motorReset), Scope/3, [HmotorResetPos]
  motorStateHandler1/3(motorResetPos) -> MATLAB Function3/1(motorReset), Scope11/1, [KmotorResetPos]
  Zero2/1 -> Manual Position Offset1/2
  motorStateHandler1/1(motorStart) -> [KmotorStart]
  motorStateHandler/2(motorStop) -> Scope/2, [HmotorStop]
  One3/1 -> Manual Position Offset2/1
  motorStateHandler/1(motorStart) -> Scope/1, [HmotorStart]
  Manual Position Offset1/1 -> motorStateHandler1/1(calibrate)
  Constant7/1 -> MATLAB Function3/2(delayTime)
  One6/1 -> Manual Position Offset4/1
  MATLAB Function3/1(delayedMotorReset) -> Scope11/2
  One2/1 -> Manual Position Offset1/1
  Zero5/1 -> Manual Position Offset3/2
  Zero6/1 -> Manual Position Offset4/2
  Manual Position Offset3/1 -> motorStateHandler/1(calibrate)
  One5/1 -> Manual Position Offset3/1
  Manual Position Offset4/1 -> motorStateHandler/2(sigma)
  Constant/1 -> MATLAB Function/2(delayTime)
  MATLAB Function/1(delayedMotorReset) -> Scope9/2

== system exo_df/MOTOR INTERFACE/CAN message dcode1/Convert 12-bit to float ==
  x_int : Inport
  x_max : Inport  Port=2
  x_min : Inport  Port=3
  Add : Sum
  Bit Shift : hdlsllib/Logic and Bit Operations/Bit Shift  Commented=on  mode=Shift Left Logical  N=12
      settings: SourceProductName=HDL Coder  SourceProductBaseCode=HD
  Constant : Constant  Value=bitshift(1,12)-1
  Divide : Product  Inputs=*/
  Product : Product
  Subtract : Sum  Inputs=+-
  Subtract1 : Sum  Commented=on  Inputs=+-
  bit : Constant  Commented=on  OutDataTypeStr=uint32
  one : Constant  Commented=on
  float : Outport  VectorParamsAs1DForOutWhenUnconnected=on
  wires:
  x_int/1 -> Product/1
  x_max/1 -> Subtract/1
  Add/1 -> float/1
  bit/1 -> Bit Shift/1
  Bit Shift/1 -> Subtract1/1
  one/1 -> Subtract1/2
  x_min/1 -> Add/2, Subtract/2
  Subtract/1 -> Product/2
  Divide/1 -> Add/1
  Product/1 -> Divide/1
  Constant/1 -> Divide/2

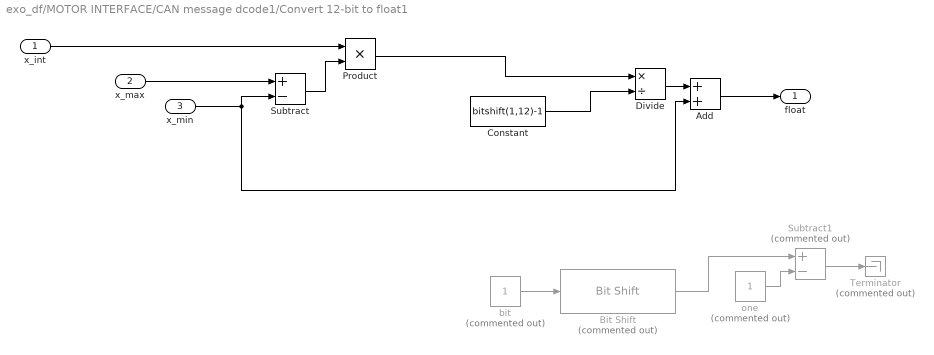
== system exo_df/MOTOR INTERFACE/CAN message dcode1/Convert 12-bit to float1 ==
  x_int : Inport
  x_max : Inport  Port=2
  x_min : Inport  Port=3
  Add : Sum
  Bit Shift : hdlsllib/Logic and Bit Operations/Bit Shift  Commented=on  mode=Shift Left Logical  N=12
      settings: SourceProductName=HDL Coder  SourceProductBaseCode=HD
  Constant : Constant  Value=bitshift(1,12)-1
  Divide : Product  Inputs=*/
  Product : Product
  Subtract : Sum  Inputs=+-
  Subtract1 : Sum  Commented=on  Inputs=+-
  Terminator : Terminator  Commented=on
  bit : Constant  Commented=on  OutDataTypeStr=uint32
  one : Constant  Commented=on
  float : Outport  VectorParamsAs1DForOutWhenUnconnected=on
  wires:
  Product/1 -> Divide/1
  Divide/1 -> Add/1
  Subtract/1 -> Product/2
  x_min/1 -> Subtract/2, Add/2
  Add/1 -> float/1
  x_max/1 -> Subtract/1
  x_int/1 -> Product/1
  one/1 -> Subtract1/2
  bit/1 -> Bit Shift/1
  Bit Shift/1 -> Subtract1/1
  Constant/1 -> Divide/2
  Subtract1/1 -> Terminator/1

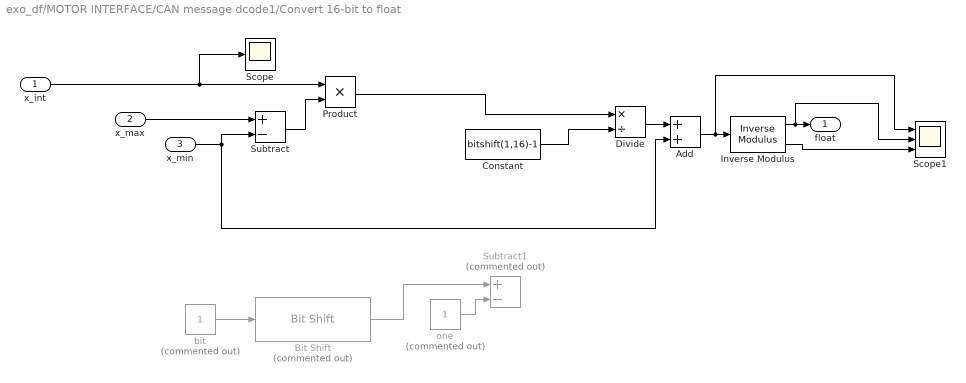
== system exo_df/MOTOR INTERFACE/CAN message dcode1/Convert 16-bit to float ==
  x_int : Inport
  x_max : Inport  Port=2
  x_min : Inport  Port=3
  Add : Sum
  Bit Shift : hdlsllib/Logic and Bit Operations/Bit Shift  Commented=on  mode=Shift Left Logical  N=16
      settings: SourceProductName=HDL Coder  SourceProductBaseCode=HD
  Constant : Constant  Value=bitshift(1,16)-1
  Divide : Product  Inputs=*/
  Inverse Modulus : quarc_library/Discontinuities/Inverse Modulus  modulus=25  output_derivative=off  output_revolutions=on  max_x=Inf  min_x=-Inf
  Product : Product
  Scope : Scope
  Scope1 : Scope  NumInputPorts=3
  Subtract : Sum  Inputs=+-
  Subtract1 : Sum  Commented=on  Inputs=+-
  bit : Constant  Commented=on  OutDataTypeStr=uint32
  one : Constant  Commented=on
  float : Outport  VectorParamsAs1DForOutWhenUnconnected=on
  wires:
  Product/1 -> Divide/1
  Divide/1 -> Add/1
  Subtract/1 -> Product/2
  x_min/1 -> Subtract/2, Add/2
  one/1 -> Subtract1/2
  Bit Shift/1 -> Subtract1/1
  bit/1 -> Bit Shift/1
  x_max/1 -> Subtract/1
  x_int/1 -> Scope/1, Product/1
  Constant/1 -> Divide/2
  Inverse Modulus/1 -> Scope1/2, float/1
  Inverse Modulus/2 -> Scope1/3
  Add/1 -> Inverse Modulus/1, Scope1/1

== system exo_df/MOTOR INTERFACE/CAN message dcode2/Convert 12-bit to float ==
  x_int : Inport
  x_max : Inport  Port=2
  x_min : Inport  Port=3
  Add : Sum
  Bit Shift : hdlsllib/Logic and Bit Operations/Bit Shift  Commented=on  mode=Shift Left Logical  N=12
      settings: SourceProductName=HDL Coder  SourceProductBaseCode=HD
  Constant : Constant  Value=bitshift(1,12)-1
  Divide : Product  Inputs=*/
  Product : Product
  Subtract : Sum  Inputs=+-
  Subtract1 : Sum  Commented=on  Inputs=+-
  bit : Constant  Commented=on  OutDataTypeStr=uint32
  one : Constant  Commented=on
  float : Outport  VectorParamsAs1DForOutWhenUnconnected=on
  wires:
  Constant/1 -> Divide/2
  Product/1 -> Divide/1
  Divide/1 -> Add/1
  Subtract/1 -> Product/2
  x_min/1 -> Subtract/2, Add/2
  one/1 -> Subtract1/2
  Bit Shift/1 -> Subtract1/1
  bit/1 -> Bit Shift/1
  Add/1 -> float/1
  x_max/1 -> Subtract/1
  x_int/1 -> Product/1

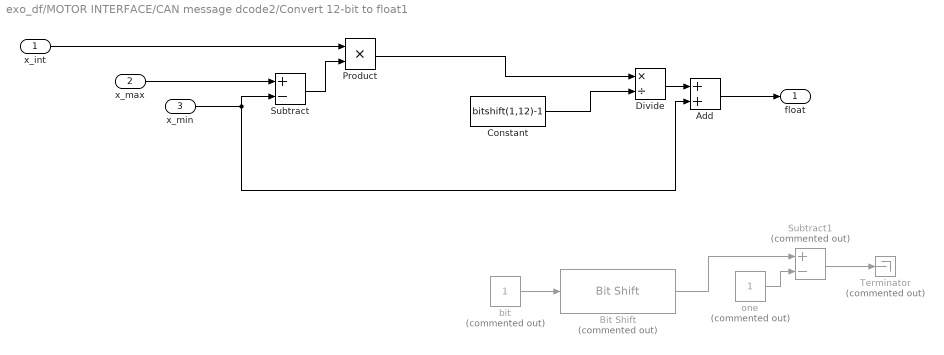
== system exo_df/MOTOR INTERFACE/CAN message dcode2/Convert 12-bit to float1 ==
  x_int : Inport
  x_max : Inport  Port=2
  x_min : Inport  Port=3
  Add : Sum
  Bit Shift : hdlsllib/Logic and Bit Operations/Bit Shift  Commented=on  mode=Shift Left Logical  N=12
      settings: SourceProductName=HDL Coder  SourceProductBaseCode=HD
  Constant : Constant  Value=bitshift(1,12)-1
  Divide : Product  Inputs=*/
  Product : Product
  Subtract : Sum  Inputs=+-
  Subtract1 : Sum  Commented=on  Inputs=+-
  Terminator : Terminator  Commented=on
  bit : Constant  Commented=on  OutDataTypeStr=uint32
  one : Constant  Commented=on
  float : Outport  VectorParamsAs1DForOutWhenUnconnected=on
  wires:
  Constant/1 -> Divide/2
  Bit Shift/1 -> Subtract1/1
  bit/1 -> Bit Shift/1
  one/1 -> Subtract1/2
  x_int/1 -> Product/1
  x_max/1 -> Subtract/1
  Add/1 -> float/1
  x_min/1 -> Add/2, Subtract/2
  Subtract/1 -> Product/2
  Divide/1 -> Add/1
  Product/1 -> Divide/1
  Subtract1/1 -> Terminator/1

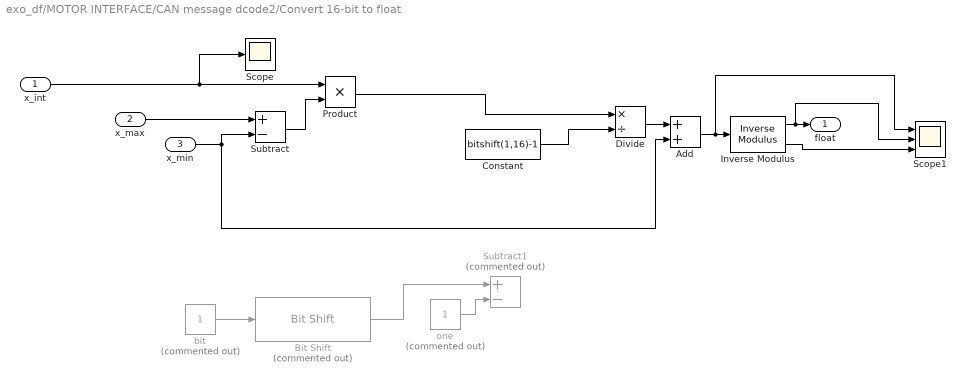
== system exo_df/MOTOR INTERFACE/CAN message dcode2/Convert 16-bit to float ==
  x_int : Inport
  x_max : Inport  Port=2
  x_min : Inport  Port=3
  Add : Sum
  Bit Shift : hdlsllib/Logic and Bit Operations/Bit Shift  Commented=on  mode=Shift Left Logical  N=16
      settings: SourceProductName=HDL Coder  SourceProductBaseCode=HD
  Constant : Constant  Value=bitshift(1,16)-1
  Divide : Product  Inputs=*/
  Inverse Modulus : quarc_library/Discontinuities/Inverse Modulus  modulus=25  output_derivative=off  output_revolutions=on  max_x=Inf  min_x=-Inf
  Product : Product
  Scope : Scope
  Scope1 : Scope  NumInputPorts=3
  Subtract : Sum  Inputs=+-
  Subtract1 : Sum  Commented=on  Inputs=+-
  bit : Constant  Commented=on  OutDataTypeStr=uint32
  one : Constant  Commented=on
  float : Outport  VectorParamsAs1DForOutWhenUnconnected=on
  wires:
  Add/1 -> Scope1/1, Inverse Modulus/1
  Inverse Modulus/2 -> Scope1/3
  Inverse Modulus/1 -> float/1, Scope1/2
  Constant/1 -> Divide/2
  x_int/1 -> Product/1, Scope/1
  x_max/1 -> Subtract/1
  bit/1 -> Bit Shift/1
  Bit Shift/1 -> Subtract1/1
  one/1 -> Subtract1/2
  x_min/1 -> Add/2, Subtract/2
  Subtract/1 -> Product/2
  Divide/1 -> Add/1
  Product/1 -> Divide/1

== system exo_df/MOTOR INTERFACE/CAN message encode/Convert float to 12-bit to float ==
  x_int : Inport
  x_max : Inport  Port=2
  x_min : Inport  Port=3
  Bit Shift : hdlsllib/Logic and Bit Operations/Bit Shift  mode=Shift Left Logical  N=12
      settings: SourceProductName=HDL Coder  SourceProductBaseCode=HD
  Data Type Conversion : DataTypeConversion  OutDataTypeStr=uint16
  Divide : Product  Inputs=*/
  Product : Product
  Subtract : Sum  Inputs=+-
  Subtract1 : Sum  Inputs=+-
  Subtract2 : Sum  Inputs=+-
  bit : Constant  OutDataTypeStr=uint32
  one : Constant
  float : Outport  VectorParamsAs1DForOutWhenUnconnected=on
  wires:
  Data Type Conversion/1 -> float/1
  Subtract2/1 -> Product/1
  x_int/1 -> Subtract2/1
  Divide/1 -> Product/2
  Subtract/1 -> Divide/2
  Subtract1/1 -> Divide/1
  x_min/1 -> Subtract/2, Subtract2/2
  one/1 -> Subtract1/2
  Bit Shift/1 -> Subtract1/1
  bit/1 -> Bit Shift/1
  Product/1 -> Data Type Conversion/1
  x_max/1 -> Subtract/1

== system exo_df/MOTOR INTERFACE/CAN message encode/Convert float to 12-bit to float1 ==
  x_int : Inport
  x_max : Inport  Port=2
  x_min : Inport  Port=3
  Bit Shift : hdlsllib/Logic and Bit Operations/Bit Shift  mode=Shift Left Logical  N=12
      settings: SourceProductName=HDL Coder  SourceProductBaseCode=HD
  Data Type Conversion : DataTypeConversion  OutDataTypeStr=uint16
  Divide : Product  Inputs=*/
  Product : Product
  Subtract : Sum  Inputs=+-
  Subtract1 : Sum  Inputs=+-
  Subtract2 : Sum  Inputs=+-
  bit : Constant  OutDataTypeStr=uint32
  one : Constant
  float : Outport  VectorParamsAs1DForOutWhenUnconnected=on
  wires:
  x_max/1 -> Subtract/1
  Product/1 -> Data Type Conversion/1
  bit/1 -> Bit Shift/1
  Bit Shift/1 -> Subtract1/1
  one/1 -> Subtract1/2
  x_min/1 -> Subtract2/2, Subtract/2
  Subtract1/1 -> Divide/1
  Subtract/1 -> Divide/2
  Divide/1 -> Product/2
  x_int/1 -> Subtract2/1
  Subtract2/1 -> Product/1
  Data Type Conversion/1 -> float/1

== system exo_df/MOTOR INTERFACE/CAN message encode/Convert float to 12-bit to float2 ==
  x_int : Inport
  x_max : Inport  Port=2
  x_min : Inport  Port=3
  Bit Shift : hdlsllib/Logic and Bit Operations/Bit Shift  mode=Shift Left Logical  N=12
      settings: SourceProductName=HDL Coder  SourceProductBaseCode=HD
  Data Type Conversion : DataTypeConversion  OutDataTypeStr=uint16
  Divide : Product  Inputs=*/
  Product : Product
  Subtract : Sum  Inputs=+-
  Subtract1 : Sum  Inputs=+-
  Subtract2 : Sum  Inputs=+-
  bit : Constant  OutDataTypeStr=uint32
  one : Constant
  float : Outport  VectorParamsAs1DForOutWhenUnconnected=on
  wires:
  x_max/1 -> Subtract/1
  Product/1 -> Data Type Conversion/1
  bit/1 -> Bit Shift/1
  Bit Shift/1 -> Subtract1/1
  one/1 -> Subtract1/2
  x_min/1 -> Subtract2/2, Subtract/2
  Subtract1/1 -> Divide/1
  Subtract/1 -> Divide/2
  Divide/1 -> Product/2
  x_int/1 -> Subtract2/1
  Subtract2/1 -> Product/1
  Data Type Conversion/1 -> float/1
